simulink library "lib_LargeBuildingModel"  (R2026a)
settings: Solver=VariableStepAuto
libraries: WallSelector_lib x380, ExternalWall_lib x188, RoomWithAirVolume x140, fl_lib x139, RoomLevelControl_lib x1
(part 5 of 12)

== system lib_LargeBuildingModel/LargeBuildingModelLib/Ground ==
  note: Ground_A1R1(LivingRoom_A)
  note: Ground_A1R2(Bedroom_A)
  note: Ground_A1R3(Kitchen_A)
  note: Ground_A1R4(Bathroom_A)
  note: Ground_A1R5(FireExit_A)
  note: Ground_A1R6(Lobby1_A)
  note: Ground_A1R7(Lobby2_A)
  note: Ground_A2R1(LivingRoom_B)
  note: Ground_A2R2(Bedroom_B)
  note: Ground_A2R3(Kitchen_B)
  note: Ground_A2R4(Bathroom_B)
  note: Ground_A2R5(FireExit_B)
  note: Ground_A2R6(Lobby1_B)
  note: Ground_A2R7(Lobby2_B)
  note: Ground_A3R1(LivingRoom_C)
  note: Ground_A3R2(Bedroom_C)
  note: Ground_A3R3(Kitchen_C)
  note: Ground_A3R4(Bathroom_C)
  note: Ground_A3R5(FireExit_C)
  note: Ground_A3R6(Lobby1_C)
  note: Ground_A3R7(Lobby2_C)
  note: Ground_A4R1(LivingRoom_D)
  note: Ground_A4R2(Bedroom_D)
  note: Ground_A4R3(Kitchen_D)
  note: Ground_A4R4(Bathroom_D)
  note: Ground_A4R5(FireExit_D)
  note: Ground_A4R6(Lobby1_D)
  note: Ground_A4R7(Lobby2_D)
  ArrayBottom : SimscapeArrayConnection  Domain=foundation.thermal.thermal  ConcatenateDimension=1  NumScalarElements=28
  ArrayTop : SimscapeArrayConnection  Domain=foundation.thermal.thermal  ConcatenateDimension=1  NumScalarElements=28
  Ground_A1R1(LivingRoom_A)Blk : WallSelector_lib/Wall Selector  optWall=wallModelOption.wallOnly  wallLength=2.4384 % Parameterized on : 13-Jun-2026 10:47:16 m  wallHeight=4.572 % Parameterized on : 13-Jun-2026 10:47:16 m  wallThickness=0.03 % Parameterized on : 13-Jun-2026 10:47:16 m  wallMaterialDen=1400 % Parameterized on : 13-Jun-2026 10:47:31 kg/m^3  wallMaterialCp=1000 % Parameterized on : 13-Jun-2026 10:47:31 J/(K*kg)  wallAbsorptivity=0.5  wallThermalK=0.7 % Parameterized on : 13-Jun-2026 10:47:31 W/(K*m)  winLength=1 m  winHeight=0.5 m  winThickness=0.007 m  winMaterialDen=2500 kg/m^3  winMaterialCp=787 J/(K*kg)  winAbsorptivity=0.35  winThermalK=1 W/(K*m)  winTransmissivity=0.45  ventLength=0.1 m  ventHeight=0.1 m  extToWallHTC=30 % Parameterized on : 13-Jun-2026 10:47:31 W/(K*m^2)  intToRoomHTC=30 % Parameterized on : 13-Jun-2026 10:47:31 W/(K*m^2)  iniT=300 % Parameterized on : 13-Jun-2026 10:47:31 K
  Ground_A1R2(Bedroom_A)Blk : WallSelector_lib/Wall Selector  optWall=wallModelOption.wallOnly  wallLength=4.2672 % Parameterized on : 13-Jun-2026 10:47:16 m  wallHeight=4.572 % Parameterized on : 13-Jun-2026 10:47:16 m  wallThickness=0.03 % Parameterized on : 13-Jun-2026 10:47:16 m  wallMaterialDen=1400 % Parameterized on : 13-Jun-2026 10:47:31 kg/m^3  wallMaterialCp=1000 % Parameterized on : 13-Jun-2026 10:47:31 J/(K*kg)  wallAbsorptivity=0.5  wallThermalK=0.7 % Parameterized on : 13-Jun-2026 10:47:31 W/(K*m)  winLength=1 m  winHeight=0.5 m  winThickness=0.007 m  winMaterialDen=2500 kg/m^3  winMaterialCp=787 J/(K*kg)  winAbsorptivity=0.35  winThermalK=1 W/(K*m)  winTransmissivity=0.45  ventLength=0.1 m  ventHeight=0.1 m  extToWallHTC=30 % Parameterized on : 13-Jun-2026 10:47:31 W/(K*m^2)  intToRoomHTC=30 % Parameterized on : 13-Jun-2026 10:47:31 W/(K*m^2)  iniT=300 % Parameterized on : 13-Jun-2026 10:47:31 K
  Ground_A1R3(Kitchen_A)Blk : WallSelector_lib/Wall Selector  optWall=wallModelOption.wallOnly  wallLength=2.7432 % Parameterized on : 13-Jun-2026 10:47:16 m  wallHeight=3.9624 % Parameterized on : 13-Jun-2026 10:47:16 m  wallThickness=0.03 % Parameterized on : 13-Jun-2026 10:47:16 m  wallMaterialDen=1400 % Parameterized on : 13-Jun-2026 10:47:31 kg/m^3  wallMaterialCp=1000 % Parameterized on : 13-Jun-2026 10:47:31 J/(K*kg)  wallAbsorptivity=0.5  wallThermalK=0.7 % Parameterized on : 13-Jun-2026 10:47:31 W/(K*m)  winLength=1 m  winHeight=0.5 m  winThickness=0.007 m  winMaterialDen=2500 kg/m^3  winMaterialCp=787 J/(K*kg)  winAbsorptivity=0.35  winThermalK=1 W/(K*m)  winTransmissivity=0.45  ventLength=0.1 m  ventHeight=0.1 m  extToWallHTC=30 % Parameterized on : 13-Jun-2026 10:47:31 W/(K*m^2)  intToRoomHTC=30 % Parameterized on : 13-Jun-2026 10:47:31 W/(K*m^2)  iniT=300 % Parameterized on : 13-Jun-2026 10:47:31 K
  Ground_A1R4(Bathroom_A)Blk : WallSelector_lib/Wall Selector  optWall=wallModelOption.wallOnly  wallLength=2.4384 % Parameterized on : 13-Jun-2026 10:47:16 m  wallHeight=3.6576 % Parameterized on : 13-Jun-2026 10:47:16 m  wallThickness=0.03 % Parameterized on : 13-Jun-2026 10:47:16 m  wallMaterialDen=1400 % Parameterized on : 13-Jun-2026 10:47:31 kg/m^3  wallMaterialCp=1000 % Parameterized on : 13-Jun-2026 10:47:31 J/(K*kg)  wallAbsorptivity=0.5  wallThermalK=0.7 % Parameterized on : 13-Jun-2026 10:47:31 W/(K*m)  winLength=1 m  winHeight=0.5 m  winThickness=0.007 m  winMaterialDen=2500 kg/m^3  winMaterialCp=787 J/(K*kg)  winAbsorptivity=0.35  winThermalK=1 W/(K*m)  winTransmissivity=0.45  ventLength=0.1 m  ventHeight=0.1 m  extToWallHTC=30 % Parameterized on : 13-Jun-2026 10:47:31 W/(K*m^2)  intToRoomHTC=30 % Parameterized on : 13-Jun-2026 10:47:31 W/(K*m^2)  iniT=300 % Parameterized on : 13-Jun-2026 10:47:31 K
  Ground_A1R5(FireExit_A)Blk : WallSelector_lib/Wall Selector  optWall=wallModelOption.wallOnly  wallLength=1.8288 % Parameterized on : 13-Jun-2026 10:47:16 m  wallHeight=2.1336 % Parameterized on : 13-Jun-2026 10:47:16 m  wallThickness=0.03 % Parameterized on : 13-Jun-2026 10:47:16 m  wallMaterialDen=1400 % Parameterized on : 13-Jun-2026 10:47:31 kg/m^3  wallMaterialCp=1000 % Parameterized on : 13-Jun-2026 10:47:31 J/(K*kg)  wallAbsorptivity=0.5  wallThermalK=0.7 % Parameterized on : 13-Jun-2026 10:47:31 W/(K*m)  winLength=1 m  winHeight=0.5 m  winThickness=0.007 m  winMaterialDen=2500 kg/m^3  winMaterialCp=787 J/(K*kg)  winAbsorptivity=0.35  winThermalK=1 W/(K*m)  winTransmissivity=0.45  ventLength=0.1 m  ventHeight=0.1 m  extToWallHTC=30 % Parameterized on : 13-Jun-2026 10:47:31 W/(K*m^2)  intToRoomHTC=30 % Parameterized on : 13-Jun-2026 10:47:31 W/(K*m^2)  iniT=300 % Parameterized on : 13-Jun-2026 10:47:31 K
  Ground_A1R6(Lobby1_A)Blk : WallSelector_lib/Wall Selector  optWall=wallModelOption.wallOnly  wallLength=2.4384 % Parameterized on : 13-Jun-2026 10:47:16 m  wallHeight=2.4384 % Parameterized on : 13-Jun-2026 10:47:16 m  wallThickness=0.03 % Parameterized on : 13-Jun-2026 10:47:16 m  wallMaterialDen=1400 % Parameterized on : 13-Jun-2026 10:47:31 kg/m^3  wallMaterialCp=1000 % Parameterized on : 13-Jun-2026 10:47:31 J/(K*kg)  wallAbsorptivity=0.5  wallThermalK=0.7 % Parameterized on : 13-Jun-2026 10:47:31 W/(K*m)  winLength=1 m  winHeight=0.5 m  winThickness=0.007 m  winMaterialDen=2500 kg/m^3  winMaterialCp=787 J/(K*kg)  winAbsorptivity=0.35  winThermalK=1 W/(K*m)  winTransmissivity=0.45  ventLength=0.1 m  ventHeight=0.1 m  extToWallHTC=30 % Parameterized on : 13-Jun-2026 10:47:31 W/(K*m^2)  intToRoomHTC=30 % Parameterized on : 13-Jun-2026 10:47:31 W/(K*m^2)  iniT=300 % Parameterized on : 13-Jun-2026 10:47:31 K
  Ground_A1R7(Lobby2_A)Blk : WallSelector_lib/Wall Selector  optWall=wallModelOption.wallOnly  wallLength=2.4384 % Parameterized on : 13-Jun-2026 10:47:16 m  wallHeight=1.524 % Parameterized on : 13-Jun-2026 10:47:16 m  wallThickness=0.03 % Parameterized on : 13-Jun-2026 10:47:16 m  wallMaterialDen=1400 % Parameterized on : 13-Jun-2026 10:47:31 kg/m^3  wallMaterialCp=1000 % Parameterized on : 13-Jun-2026 10:47:31 J/(K*kg)  wallAbsorptivity=0.5  wallThermalK=0.7 % Parameterized on : 13-Jun-2026 10:47:31 W/(K*m)  winLength=1 m  winHeight=0.5 m  winThickness=0.007 m  winMaterialDen=2500 kg/m^3  winMaterialCp=787 J/(K*kg)  winAbsorptivity=0.35  winThermalK=1 W/(K*m)  winTransmissivity=0.45  ventLength=0.1 m  ventHeight=0.1 m  extToWallHTC=30 % Parameterized on : 13-Jun-2026 10:47:31 W/(K*m^2)  intToRoomHTC=30 % Parameterized on : 13-Jun-2026 10:47:31 W/(K*m^2)  iniT=300 % Parameterized on : 13-Jun-2026 10:47:31 K
  Ground_A2R1(LivingRoom_B)Blk : WallSelector_lib/Wall Selector  optWall=wallModelOption.wallOnly  wallLength=2.4384 % Parameterized on : 13-Jun-2026 10:47:16 m  wallHeight=4.572 % Parameterized on : 13-Jun-2026 10:47:16 m  wallThickness=0.03 % Parameterized on : 13-Jun-2026 10:47:16 m  wallMaterialDen=1400 % Parameterized on : 13-Jun-2026 10:47:31 kg/m^3  wallMaterialCp=1000 % Parameterized on : 13-Jun-2026 10:47:31 J/(K*kg)  wallAbsorptivity=0.5  wallThermalK=0.7 % Parameterized on : 13-Jun-2026 10:47:31 W/(K*m)  winLength=1 m  winHeight=0.5 m  winThickness=0.007 m  winMaterialDen=2500 kg/m^3  winMaterialCp=787 J/(K*kg)  winAbsorptivity=0.35  winThermalK=1 W/(K*m)  winTransmissivity=0.45  ventLength=0.1 m  ventHeight=0.1 m  extToWallHTC=30 % Parameterized on : 13-Jun-2026 10:47:31 W/(K*m^2)  intToRoomHTC=30 % Parameterized on : 13-Jun-2026 10:47:31 W/(K*m^2)  iniT=300 % Parameterized on : 13-Jun-2026 10:47:31 K
  Ground_A2R2(Bedroom_B)Blk : WallSelector_lib/Wall Selector  optWall=wallModelOption.wallOnly  wallLength=4.2672 % Parameterized on : 13-Jun-2026 10:47:16 m  wallHeight=4.572 % Parameterized on : 13-Jun-2026 10:47:16 m  wallThickness=0.03 % Parameterized on : 13-Jun-2026 10:47:16 m  wallMaterialDen=1400 % Parameterized on : 13-Jun-2026 10:47:31 kg/m^3  wallMaterialCp=1000 % Parameterized on : 13-Jun-2026 10:47:31 J/(K*kg)  wallAbsorptivity=0.5  wallThermalK=0.7 % Parameterized on : 13-Jun-2026 10:47:31 W/(K*m)  winLength=1 m  winHeight=0.5 m  winThickness=0.007 m  winMaterialDen=2500 kg/m^3  winMaterialCp=787 J/(K*kg)  winAbsorptivity=0.35  winThermalK=1 W/(K*m)  winTransmissivity=0.45  ventLength=0.1 m  ventHeight=0.1 m  extToWallHTC=30 % Parameterized on : 13-Jun-2026 10:47:31 W/(K*m^2)  intToRoomHTC=30 % Parameterized on : 13-Jun-2026 10:47:31 W/(K*m^2)  iniT=300 % Parameterized on : 13-Jun-2026 10:47:31 K
  Ground_A2R3(Kitchen_B)Blk : WallSelector_lib/Wall Selector  optWall=wallModelOption.wallOnly  wallLength=2.7432 % Parameterized on : 13-Jun-2026 10:47:16 m  wallHeight=3.9624 % Parameterized on : 13-Jun-2026 10:47:16 m  wallThickness=0.03 % Parameterized on : 13-Jun-2026 10:47:16 m  wallMaterialDen=1400 % Parameterized on : 13-Jun-2026 10:47:31 kg/m^3  wallMaterialCp=1000 % Parameterized on : 13-Jun-2026 10:47:31 J/(K*kg)  wallAbsorptivity=0.5  wallThermalK=0.7 % Parameterized on : 13-Jun-2026 10:47:31 W/(K*m)  winLength=1 m  winHeight=0.5 m  winThickness=0.007 m  winMaterialDen=2500 kg/m^3  winMaterialCp=787 J/(K*kg)  winAbsorptivity=0.35  winThermalK=1 W/(K*m)  winTransmissivity=0.45  ventLength=0.1 m  ventHeight=0.1 m  extToWallHTC=30 % Parameterized on : 13-Jun-2026 10:47:31 W/(K*m^2)  intToRoomHTC=30 % Parameterized on : 13-Jun-2026 10:47:31 W/(K*m^2)  iniT=300 % Parameterized on : 13-Jun-2026 10:47:31 K
  Ground_A2R4(Bathroom_B)Blk : WallSelector_lib/Wall Selector  optWall=wallModelOption.wallOnly  wallLength=2.4384 % Parameterized on : 13-Jun-2026 10:47:16 m  wallHeight=3.6576 % Parameterized on : 13-Jun-2026 10:47:16 m  wallThickness=0.03 % Parameterized on : 13-Jun-2026 10:47:16 m  wallMaterialDen=1400 % Parameterized on : 13-Jun-2026 10:47:31 kg/m^3  wallMaterialCp=1000 % Parameterized on : 13-Jun-2026 10:47:31 J/(K*kg)  wallAbsorptivity=0.5  wallThermalK=0.7 % Parameterized on : 13-Jun-2026 10:47:31 W/(K*m)  winLength=1 m  winHeight=0.5 m  winThickness=0.007 m  winMaterialDen=2500 kg/m^3  winMaterialCp=787 J/(K*kg)  winAbsorptivity=0.35  winThermalK=1 W/(K*m)  winTransmissivity=0.45  ventLength=0.1 m  ventHeight=0.1 m  extToWallHTC=30 % Parameterized on : 13-Jun-2026 10:47:31 W/(K*m^2)  intToRoomHTC=30 % Parameterized on : 13-Jun-2026 10:47:31 W/(K*m^2)  iniT=300 % Parameterized on : 13-Jun-2026 10:47:31 K
  Ground_A2R5(FireExit_B)Blk : WallSelector_lib/Wall Selector  optWall=wallModelOption.wallOnly  wallLength=1.8288 % Parameterized on : 13-Jun-2026 10:47:16 m  wallHeight=2.1336 % Parameterized on : 13-Jun-2026 10:47:16 m  wallThickness=0.03 % Parameterized on : 13-Jun-2026 10:47:16 m  wallMaterialDen=1400 % Parameterized on : 13-Jun-2026 10:47:31 kg/m^3  wallMaterialCp=1000 % Parameterized on : 13-Jun-2026 10:47:31 J/(K*kg)  wallAbsorptivity=0.5  wallThermalK=0.7 % Parameterized on : 13-Jun-2026 10:47:31 W/(K*m)  winLength=1 m  winHeight=0.5 m  winThickness=0.007 m  winMaterialDen=2500 kg/m^3  winMaterialCp=787 J/(K*kg)  winAbsorptivity=0.35  winThermalK=1 W/(K*m)  winTransmissivity=0.45  ventLength=0.1 m  ventHeight=0.1 m  extToWallHTC=30 % Parameterized on : 13-Jun-2026 10:47:31 W/(K*m^2)  intToRoomHTC=30 % Parameterized on : 13-Jun-2026 10:47:31 W/(K*m^2)  iniT=300 % Parameterized on : 13-Jun-2026 10:47:31 K
  Ground_A2R6(Lobby1_B)Blk : WallSelector_lib/Wall Selector  optWall=wallModelOption.wallOnly  wallLength=2.4384 % Parameterized on : 13-Jun-2026 10:47:16 m  wallHeight=2.4384 % Parameterized on : 13-Jun-2026 10:47:16 m  wallThickness=0.03 % Parameterized on : 13-Jun-2026 10:47:16 m  wallMaterialDen=1400 % Parameterized on : 13-Jun-2026 10:47:31 kg/m^3  wallMaterialCp=1000 % Parameterized on : 13-Jun-2026 10:47:31 J/(K*kg)  wallAbsorptivity=0.5  wallThermalK=0.7 % Parameterized on : 13-Jun-2026 10:47:31 W/(K*m)  winLength=1 m  winHeight=0.5 m  winThickness=0.007 m  winMaterialDen=2500 kg/m^3  winMaterialCp=787 J/(K*kg)  winAbsorptivity=0.35  winThermalK=1 W/(K*m)  winTransmissivity=0.45  ventLength=0.1 m  ventHeight=0.1 m  extToWallHTC=30 % Parameterized on : 13-Jun-2026 10:47:31 W/(K*m^2)  intToRoomHTC=30 % Parameterized on : 13-Jun-2026 10:47:31 W/(K*m^2)  iniT=300 % Parameterized on : 13-Jun-2026 10:47:31 K
  Ground_A2R7(Lobby2_B)Blk : WallSelector_lib/Wall Selector  optWall=wallModelOption.wallOnly  wallLength=2.4384 % Parameterized on : 13-Jun-2026 10:47:16 m  wallHeight=1.524 % Parameterized on : 13-Jun-2026 10:47:16 m  wallThickness=0.03 % Parameterized on : 13-Jun-2026 10:47:16 m  wallMaterialDen=1400 % Parameterized on : 13-Jun-2026 10:47:31 kg/m^3  wallMaterialCp=1000 % Parameterized on : 13-Jun-2026 10:47:31 J/(K*kg)  wallAbsorptivity=0.5  wallThermalK=0.7 % Parameterized on : 13-Jun-2026 10:47:31 W/(K*m)  winLength=1 m  winHeight=0.5 m  winThickness=0.007 m  winMaterialDen=2500 kg/m^3  winMaterialCp=787 J/(K*kg)  winAbsorptivity=0.35  winThermalK=1 W/(K*m)  winTransmissivity=0.45  ventLength=0.1 m  ventHeight=0.1 m  extToWallHTC=30 % Parameterized on : 13-Jun-2026 10:47:31 W/(K*m^2)  intToRoomHTC=30 % Parameterized on : 13-Jun-2026 10:47:31 W/(K*m^2)  iniT=300 % Parameterized on : 13-Jun-2026 10:47:31 K
  Ground_A3R1(LivingRoom_C)Blk : WallSelector_lib/Wall Selector  optWall=wallModelOption.wallOnly  wallLength=2.4384 % Parameterized on : 13-Jun-2026 10:47:16 m  wallHeight=4.572 % Parameterized on : 13-Jun-2026 10:47:16 m  wallThickness=0.03 % Parameterized on : 13-Jun-2026 10:47:16 m  wallMaterialDen=1400 % Parameterized on : 13-Jun-2026 10:47:31 kg/m^3  wallMaterialCp=1000 % Parameterized on : 13-Jun-2026 10:47:31 J/(K*kg)  wallAbsorptivity=0.5  wallThermalK=0.7 % Parameterized on : 13-Jun-2026 10:47:31 W/(K*m)  winLength=1 m  winHeight=0.5 m  winThickness=0.007 m  winMaterialDen=2500 kg/m^3  winMaterialCp=787 J/(K*kg)  winAbsorptivity=0.35  winThermalK=1 W/(K*m)  winTransmissivity=0.45  ventLength=0.1 m  ventHeight=0.1 m  extToWallHTC=30 % Parameterized on : 13-Jun-2026 10:47:31 W/(K*m^2)  intToRoomHTC=30 % Parameterized on : 13-Jun-2026 10:47:31 W/(K*m^2)  iniT=300 % Parameterized on : 13-Jun-2026 10:47:31 K
  Ground_A3R2(Bedroom_C)Blk : WallSelector_lib/Wall Selector  optWall=wallModelOption.wallOnly  wallLength=4.2672 % Parameterized on : 13-Jun-2026 10:47:16 m  wallHeight=4.572 % Parameterized on : 13-Jun-2026 10:47:16 m  wallThickness=0.03 % Parameterized on : 13-Jun-2026 10:47:16 m  wallMaterialDen=1400 % Parameterized on : 13-Jun-2026 10:47:31 kg/m^3  wallMaterialCp=1000 % Parameterized on : 13-Jun-2026 10:47:31 J/(K*kg)  wallAbsorptivity=0.5  wallThermalK=0.7 % Parameterized on : 13-Jun-2026 10:47:31 W/(K*m)  winLength=1 m  winHeight=0.5 m  winThickness=0.007 m  winMaterialDen=2500 kg/m^3  winMaterialCp=787 J/(K*kg)  winAbsorptivity=0.35  winThermalK=1 W/(K*m)  winTransmissivity=0.45  ventLength=0.1 m  ventHeight=0.1 m  extToWallHTC=30 % Parameterized on : 13-Jun-2026 10:47:31 W/(K*m^2)  intToRoomHTC=30 % Parameterized on : 13-Jun-2026 10:47:31 W/(K*m^2)  iniT=300 % Parameterized on : 13-Jun-2026 10:47:31 K
  Ground_A3R3(Kitchen_C)Blk : WallSelector_lib/Wall Selector  optWall=wallModelOption.wallOnly  wallLength=2.7432 % Parameterized on : 13-Jun-2026 10:47:16 m  wallHeight=3.9624 % Parameterized on : 13-Jun-2026 10:47:16 m  wallThickness=0.03 % Parameterized on : 13-Jun-2026 10:47:16 m  wallMaterialDen=1400 % Parameterized on : 13-Jun-2026 10:47:31 kg/m^3  wallMaterialCp=1000 % Parameterized on : 13-Jun-2026 10:47:31 J/(K*kg)  wallAbsorptivity=0.5  wallThermalK=0.7 % Parameterized on : 13-Jun-2026 10:47:31 W/(K*m)  winLength=1 m  winHeight=0.5 m  winThickness=0.007 m  winMaterialDen=2500 kg/m^3  winMaterialCp=787 J/(K*kg)  winAbsorptivity=0.35  winThermalK=1 W/(K*m)  winTransmissivity=0.45  ventLength=0.1 m  ventHeight=0.1 m  extToWallHTC=30 % Parameterized on : 13-Jun-2026 10:47:31 W/(K*m^2)  intToRoomHTC=30 % Parameterized on : 13-Jun-2026 10:47:31 W/(K*m^2)  iniT=300 % Parameterized on : 13-Jun-2026 10:47:31 K
  Ground_A3R4(Bathroom_C)Blk : WallSelector_lib/Wall Selector  optWall=wallModelOption.wallOnly  wallLength=2.4384 % Parameterized on : 13-Jun-2026 10:47:16 m  wallHeight=3.6576 % Parameterized on : 13-Jun-2026 10:47:16 m  wallThickness=0.03 % Parameterized on : 13-Jun-2026 10:47:16 m  wallMaterialDen=1400 % Parameterized on : 13-Jun-2026 10:47:31 kg/m^3  wallMaterialCp=1000 % Parameterized on : 13-Jun-2026 10:47:31 J/(K*kg)  wallAbsorptivity=0.5  wallThermalK=0.7 % Parameterized on : 13-Jun-2026 10:47:31 W/(K*m)  winLength=1 m  winHeight=0.5 m  winThickness=0.007 m  winMaterialDen=2500 kg/m^3  winMaterialCp=787 J/(K*kg)  winAbsorptivity=0.35  winThermalK=1 W/(K*m)  winTransmissivity=0.45  ventLength=0.1 m  ventHeight=0.1 m  extToWallHTC=30 % Parameterized on : 13-Jun-2026 10:47:31 W/(K*m^2)  intToRoomHTC=30 % Parameterized on : 13-Jun-2026 10:47:31 W/(K*m^2)  iniT=300 % Parameterized on : 13-Jun-2026 10:47:31 K
  Ground_A3R5(FireExit_C)Blk : WallSelector_lib/Wall Selector  optWall=wallModelOption.wallOnly  wallLength=1.8288 % Parameterized on : 13-Jun-2026 10:47:16 m  wallHeight=2.1336 % Parameterized on : 13-Jun-2026 10:47:16 m  wallThickness=0.03 % Parameterized on : 13-Jun-2026 10:47:16 m  wallMaterialDen=1400 % Parameterized on : 13-Jun-2026 10:47:31 kg/m^3  wallMaterialCp=1000 % Parameterized on : 13-Jun-2026 10:47:31 J/(K*kg)  wallAbsorptivity=0.5  wallThermalK=0.7 % Parameterized on : 13-Jun-2026 10:47:31 W/(K*m)  winLength=1 m  winHeight=0.5 m  winThickness=0.007 m  winMaterialDen=2500 kg/m^3  winMaterialCp=787 J/(K*kg)  winAbsorptivity=0.35  winThermalK=1 W/(K*m)  winTransmissivity=0.45  ventLength=0.1 m  ventHeight=0.1 m  extToWallHTC=30 % Parameterized on : 13-Jun-2026 10:47:31 W/(K*m^2)  intToRoomHTC=30 % Parameterized on : 13-Jun-2026 10:47:31 W/(K*m^2)  iniT=300 % Parameterized on : 13-Jun-2026 10:47:31 K
  Ground_A3R6(Lobby1_C)Blk : WallSelector_lib/Wall Selector  optWall=wallModelOption.wallOnly  wallLength=2.4384 % Parameterized on : 13-Jun-2026 10:47:16 m  wallHeight=2.4384 % Parameterized on : 13-Jun-2026 10:47:16 m  wallThickness=0.03 % Parameterized on : 13-Jun-2026 10:47:16 m  wallMaterialDen=1400 % Parameterized on : 13-Jun-2026 10:47:31 kg/m^3  wallMaterialCp=1000 % Parameterized on : 13-Jun-2026 10:47:31 J/(K*kg)  wallAbsorptivity=0.5  wallThermalK=0.7 % Parameterized on : 13-Jun-2026 10:47:31 W/(K*m)  winLength=1 m  winHeight=0.5 m  winThickness=0.007 m  winMaterialDen=2500 kg/m^3  winMaterialCp=787 J/(K*kg)  winAbsorptivity=0.35  winThermalK=1 W/(K*m)  winTransmissivity=0.45  ventLength=0.1 m  ventHeight=0.1 m  extToWallHTC=30 % Parameterized on : 13-Jun-2026 10:47:31 W/(K*m^2)  intToRoomHTC=30 % Parameterized on : 13-Jun-2026 10:47:31 W/(K*m^2)  iniT=300 % Parameterized on : 13-Jun-2026 10:47:31 K
  Ground_A3R7(Lobby2_C)Blk : WallSelector_lib/Wall Selector  optWall=wallModelOption.wallOnly  wallLength=2.4384 % Parameterized on : 13-Jun-2026 10:47:16 m  wallHeight=1.524 % Parameterized on : 13-Jun-2026 10:47:16 m  wallThickness=0.03 % Parameterized on : 13-Jun-2026 10:47:16 m  wallMaterialDen=1400 % Parameterized on : 13-Jun-2026 10:47:31 kg/m^3  wallMaterialCp=1000 % Parameterized on : 13-Jun-2026 10:47:31 J/(K*kg)  wallAbsorptivity=0.5  wallThermalK=0.7 % Parameterized on : 13-Jun-2026 10:47:31 W/(K*m)  winLength=1 m  winHeight=0.5 m  winThickness=0.007 m  winMaterialDen=2500 kg/m^3  winMaterialCp=787 J/(K*kg)  winAbsorptivity=0.35  winThermalK=1 W/(K*m)  winTransmissivity=0.45  ventLength=0.1 m  ventHeight=0.1 m  extToWallHTC=30 % Parameterized on : 13-Jun-2026 10:47:31 W/(K*m^2)  intToRoomHTC=30 % Parameterized on : 13-Jun-2026 10:47:31 W/(K*m^2)  iniT=300 % Parameterized on : 13-Jun-2026 10:47:31 K
  Ground_A4R1(LivingRoom_D)Blk : WallSelector_lib/Wall Selector  optWall=wallModelOption.wallOnly  wallLength=2.4384 % Parameterized on : 13-Jun-2026 10:47:16 m  wallHeight=4.572 % Parameterized on : 13-Jun-2026 10:47:16 m  wallThickness=0.03 % Parameterized on : 13-Jun-2026 10:47:16 m  wallMaterialDen=1400 % Parameterized on : 13-Jun-2026 10:47:31 kg/m^3  wallMaterialCp=1000 % Parameterized on : 13-Jun-2026 10:47:31 J/(K*kg)  wallAbsorptivity=0.5  wallThermalK=0.7 % Parameterized on : 13-Jun-2026 10:47:31 W/(K*m)  winLength=1 m  winHeight=0.5 m  winThickness=0.007 m  winMaterialDen=2500 kg/m^3  winMaterialCp=787 J/(K*kg)  winAbsorptivity=0.35  winThermalK=1 W/(K*m)  winTransmissivity=0.45  ventLength=0.1 m  ventHeight=0.1 m  extToWallHTC=30 % Parameterized on : 13-Jun-2026 10:47:31 W/(K*m^2)  intToRoomHTC=30 % Parameterized on : 13-Jun-2026 10:47:31 W/(K*m^2)  iniT=300 % Parameterized on : 13-Jun-2026 10:47:31 K
  Ground_A4R2(Bedroom_D)Blk : WallSelector_lib/Wall Selector  optWall=wallModelOption.wallOnly  wallLength=4.2672 % Parameterized on : 13-Jun-2026 10:47:16 m  wallHeight=4.572 % Parameterized on : 13-Jun-2026 10:47:16 m  wallThickness=0.03 % Parameterized on : 13-Jun-2026 10:47:16 m  wallMaterialDen=1400 % Parameterized on : 13-Jun-2026 10:47:31 kg/m^3  wallMaterialCp=1000 % Parameterized on : 13-Jun-2026 10:47:31 J/(K*kg)  wallAbsorptivity=0.5  wallThermalK=0.7 % Parameterized on : 13-Jun-2026 10:47:31 W/(K*m)  winLength=1 m  winHeight=0.5 m  winThickness=0.007 m  winMaterialDen=2500 kg/m^3  winMaterialCp=787 J/(K*kg)  winAbsorptivity=0.35  winThermalK=1 W/(K*m)  winTransmissivity=0.45  ventLength=0.1 m  ventHeight=0.1 m  extToWallHTC=30 % Parameterized on : 13-Jun-2026 10:47:31 W/(K*m^2)  intToRoomHTC=30 % Parameterized on : 13-Jun-2026 10:47:31 W/(K*m^2)  iniT=300 % Parameterized on : 13-Jun-2026 10:47:31 K
  Ground_A4R3(Kitchen_D)Blk : WallSelector_lib/Wall Selector  optWall=wallModelOption.wallOnly  wallLength=2.7432 % Parameterized on : 13-Jun-2026 10:47:16 m  wallHeight=3.9624 % Parameterized on : 13-Jun-2026 10:47:16 m  wallThickness=0.03 % Parameterized on : 13-Jun-2026 10:47:16 m  wallMaterialDen=1400 % Parameterized on : 13-Jun-2026 10:47:31 kg/m^3  wallMaterialCp=1000 % Parameterized on : 13-Jun-2026 10:47:31 J/(K*kg)  wallAbsorptivity=0.5  wallThermalK=0.7 % Parameterized on : 13-Jun-2026 10:47:31 W/(K*m)  winLength=1 m  winHeight=0.5 m  winThickness=0.007 m  winMaterialDen=2500 kg/m^3  winMaterialCp=787 J/(K*kg)  winAbsorptivity=0.35  winThermalK=1 W/(K*m)  winTransmissivity=0.45  ventLength=0.1 m  ventHeight=0.1 m  extToWallHTC=30 % Parameterized on : 13-Jun-2026 10:47:31 W/(K*m^2)  intToRoomHTC=30 % Parameterized on : 13-Jun-2026 10:47:31 W/(K*m^2)  iniT=300 % Parameterized on : 13-Jun-2026 10:47:31 K
  Ground_A4R4(Bathroom_D)Blk : WallSelector_lib/Wall Selector  optWall=wallModelOption.wallOnly  wallLength=2.4384 % Parameterized on : 13-Jun-2026 10:47:16 m  wallHeight=3.6576 % Parameterized on : 13-Jun-2026 10:47:16 m  wallThickness=0.03 % Parameterized on : 13-Jun-2026 10:47:16 m  wallMaterialDen=1400 % Parameterized on : 13-Jun-2026 10:47:31 kg/m^3  wallMaterialCp=1000 % Parameterized on : 13-Jun-2026 10:47:31 J/(K*kg)  wallAbsorptivity=0.5  wallThermalK=0.7 % Parameterized on : 13-Jun-2026 10:47:31 W/(K*m)  winLength=1 m  winHeight=0.5 m  winThickness=0.007 m  winMaterialDen=2500 kg/m^3  winMaterialCp=787 J/(K*kg)  winAbsorptivity=0.35  winThermalK=1 W/(K*m)  winTransmissivity=0.45  ventLength=0.1 m  ventHeight=0.1 m  extToWallHTC=30 % Parameterized on : 13-Jun-2026 10:47:31 W/(K*m^2)  intToRoomHTC=30 % Parameterized on : 13-Jun-2026 10:47:31 W/(K*m^2)  iniT=300 % Parameterized on : 13-Jun-2026 10:47:31 K
  Ground_A4R5(FireExit_D)Blk : WallSelector_lib/Wall Selector  optWall=wallModelOption.wallOnly  wallLength=1.8288 % Parameterized on : 13-Jun-2026 10:47:16 m  wallHeight=2.1336 % Parameterized on : 13-Jun-2026 10:47:16 m  wallThickness=0.03 % Parameterized on : 13-Jun-2026 10:47:16 m  wallMaterialDen=1400 % Parameterized on : 13-Jun-2026 10:47:31 kg/m^3  wallMaterialCp=1000 % Parameterized on : 13-Jun-2026 10:47:31 J/(K*kg)  wallAbsorptivity=0.5  wallThermalK=0.7 % Parameterized on : 13-Jun-2026 10:47:31 W/(K*m)  winLength=1 m  winHeight=0.5 m  winThickness=0.007 m  winMaterialDen=2500 kg/m^3  winMaterialCp=787 J/(K*kg)  winAbsorptivity=0.35  winThermalK=1 W/(K*m)  winTransmissivity=0.45  ventLength=0.1 m  ventHeight=0.1 m  extToWallHTC=30 % Parameterized on : 13-Jun-2026 10:47:31 W/(K*m^2)  intToRoomHTC=30 % Parameterized on : 13-Jun-2026 10:47:31 W/(K*m^2)  iniT=300 % Parameterized on : 13-Jun-2026 10:47:31 K
  Ground_A4R6(Lobby1_D)Blk : WallSelector_lib/Wall Selector  optWall=wallModelOption.wallOnly  wallLength=2.4384 % Parameterized on : 13-Jun-2026 10:47:16 m  wallHeight=2.4384 % Parameterized on : 13-Jun-2026 10:47:16 m  wallThickness=0.03 % Parameterized on : 13-Jun-2026 10:47:16 m  wallMaterialDen=1400 % Parameterized on : 13-Jun-2026 10:47:31 kg/m^3  wallMaterialCp=1000 % Parameterized on : 13-Jun-2026 10:47:31 J/(K*kg)  wallAbsorptivity=0.5  wallThermalK=0.7 % Parameterized on : 13-Jun-2026 10:47:31 W/(K*m)  winLength=1 m  winHeight=0.5 m  winThickness=0.007 m  winMaterialDen=2500 kg/m^3  winMaterialCp=787 J/(K*kg)  winAbsorptivity=0.35  winThermalK=1 W/(K*m)  winTransmissivity=0.45  ventLength=0.1 m  ventHeight=0.1 m  extToWallHTC=30 % Parameterized on : 13-Jun-2026 10:47:31 W/(K*m^2)  intToRoomHTC=30 % Parameterized on : 13-Jun-2026 10:47:31 W/(K*m^2)  iniT=300 % Parameterized on : 13-Jun-2026 10:47:31 K
  Ground_A4R7(Lobby2_D)Blk : WallSelector_lib/Wall Selector  optWall=wallModelOption.wallOnly  wallLength=2.4384 % Parameterized on : 13-Jun-2026 10:47:16 m  wallHeight=1.524 % Parameterized on : 13-Jun-2026 10:47:16 m  wallThickness=0.03 % Parameterized on : 13-Jun-2026 10:47:16 m  wallMaterialDen=1400 % Parameterized on : 13-Jun-2026 10:47:31 kg/m^3  wallMaterialCp=1000 % Parameterized on : 13-Jun-2026 10:47:31 J/(K*kg)  wallAbsorptivity=0.5  wallThermalK=0.7 % Parameterized on : 13-Jun-2026 10:47:31 W/(K*m)  winLength=1 m  winHeight=0.5 m  winThickness=0.007 m  winMaterialDen=2500 kg/m^3  winMaterialCp=787 J/(K*kg)  winAbsorptivity=0.35  winThermalK=1 W/(K*m)  winTransmissivity=0.45  ventLength=0.1 m  ventHeight=0.1 m  extToWallHTC=30 % Parameterized on : 13-Jun-2026 10:47:31 W/(K*m^2)  intToRoomHTC=30 % Parameterized on : 13-Jun-2026 10:47:31 W/(K*m^2)  iniT=300 % Parameterized on : 13-Jun-2026 10:47:31 K
  Top : PMIOPort  Side=Left
  Bottom : PMIOPort  Port=2  Side=Right
  connections:
  ArrayTop/RConn1 -- Top/RConn1
  Ground_A1R1(LivingRoom_A)Blk/LConn1 -- ArrayTop/LConn1
  Ground_A1R2(Bedroom_A)Blk/LConn1 -- ArrayTop/LConn2
  Ground_A1R3(Kitchen_A)Blk/LConn1 -- ArrayTop/LConn3
  Ground_A1R4(Bathroom_A)Blk/LConn1 -- ArrayTop/LConn4
  Ground_A1R5(FireExit_A)Blk/LConn1 -- ArrayTop/LConn5
  Ground_A1R6(Lobby1_A)Blk/LConn1 -- ArrayTop/LConn6
  Ground_A1R7(Lobby2_A)Blk/LConn1 -- ArrayTop/LConn7
  Ground_A2R1(LivingRoom_B)Blk/LConn1 -- ArrayTop/LConn8
  Ground_A2R2(Bedroom_B)Blk/LConn1 -- ArrayTop/LConn9
  Ground_A2R3(Kitchen_B)Blk/LConn1 -- ArrayTop/LConn10
  Ground_A2R4(Bathroom_B)Blk/LConn1 -- ArrayTop/LConn11
  Ground_A2R5(FireExit_B)Blk/LConn1 -- ArrayTop/LConn12
  Ground_A2R6(Lobby1_B)Blk/LConn1 -- ArrayTop/LConn13
  Ground_A2R7(Lobby2_B)Blk/LConn1 -- ArrayTop/LConn14
  Ground_A3R1(LivingRoom_C)Blk/LConn1 -- ArrayTop/LConn15
  Ground_A3R2(Bedroom_C)Blk/LConn1 -- ArrayTop/LConn16
  Ground_A3R3(Kitchen_C)Blk/LConn1 -- ArrayTop/LConn17
  Ground_A3R4(Bathroom_C)Blk/LConn1 -- ArrayTop/LConn18
  Ground_A3R5(FireExit_C)Blk/LConn1 -- ArrayTop/LConn19
  Ground_A3R6(Lobby1_C)Blk/LConn1 -- ArrayTop/LConn20
  Ground_A3R7(Lobby2_C)Blk/LConn1 -- ArrayTop/LConn21
  Ground_A4R1(LivingRoom_D)Blk/LConn1 -- ArrayTop/LConn22
  Ground_A4R2(Bedroom_D)Blk/LConn1 -- ArrayTop/LConn23
  Ground_A4R3(Kitchen_D)Blk/LConn1 -- ArrayTop/LConn24
  Ground_A4R4(Bathroom_D)Blk/LConn1 -- ArrayTop/LConn25
  Ground_A4R5(FireExit_D)Blk/LConn1 -- ArrayTop/LConn26
  Ground_A4R6(Lobby1_D)Blk/LConn1 -- ArrayTop/LConn27
  Ground_A4R7(Lobby2_D)Blk/LConn1 -- ArrayTop/LConn28
  ArrayBottom/RConn1 -- Bottom/RConn1
  Ground_A1R1(LivingRoom_A)Blk/RConn1 -- ArrayBottom/LConn1
  Ground_A1R2(Bedroom_A)Blk/RConn1 -- ArrayBottom/LConn2
  Ground_A1R3(Kitchen_A)Blk/RConn1 -- ArrayBottom/LConn3
  Ground_A1R4(Bathroom_A)Blk/RConn1 -- ArrayBottom/LConn4
  Ground_A1R5(FireExit_A)Blk/RConn1 -- ArrayBottom/LConn5
  Ground_A1R6(Lobby1_A)Blk/RConn1 -- ArrayBottom/LConn6
  Ground_A1R7(Lobby2_A)Blk/RConn1 -- ArrayBottom/LConn7
  Ground_A2R1(LivingRoom_B)Blk/RConn1 -- ArrayBottom/LConn8
  Ground_A2R2(Bedroom_B)Blk/RConn1 -- ArrayBottom/LConn9
  Ground_A2R3(Kitchen_B)Blk/RConn1 -- ArrayBottom/LConn10
  Ground_A2R4(Bathroom_B)Blk/RConn1 -- ArrayBottom/LConn11
  Ground_A2R5(FireExit_B)Blk/RConn1 -- ArrayBottom/LConn12
  Ground_A2R6(Lobby1_B)Blk/RConn1 -- ArrayBottom/LConn13
  Ground_A2R7(Lobby2_B)Blk/RConn1 -- ArrayBottom/LConn14
  Ground_A3R1(LivingRoom_C)Blk/RConn1 -- ArrayBottom/LConn15
  Ground_A3R2(Bedroom_C)Blk/RConn1 -- ArrayBottom/LConn16
  Ground_A3R3(Kitchen_C)Blk/RConn1 -- ArrayBottom/LConn17
  Ground_A3R4(Bathroom_C)Blk/RConn1 -- ArrayBottom/LConn18
  Ground_A3R5(FireExit_C)Blk/RConn1 -- ArrayBottom/LConn19
  Ground_A3R6(Lobby1_C)Blk/RConn1 -- ArrayBottom/LConn20
  Ground_A3R7(Lobby2_C)Blk/RConn1 -- ArrayBottom/LConn21
  Ground_A4R1(LivingRoom_D)Blk/RConn1 -- ArrayBottom/LConn22
  Ground_A4R2(Bedroom_D)Blk/RConn1 -- ArrayBottom/LConn23
  Ground_A4R3(Kitchen_D)Blk/RConn1 -- ArrayBottom/LConn24
  Ground_A4R4(Bathroom_D)Blk/RConn1 -- ArrayBottom/LConn25
  Ground_A4R5(FireExit_D)Blk/RConn1 -- ArrayBottom/LConn26
  Ground_A4R6(Lobby1_D)Blk/RConn1 -- ArrayBottom/LConn27
  Ground_A4R7(Lobby2_D)Blk/RConn1 -- ArrayBottom/LConn28
